simulink library "Model_GridElem_Arc_Fault"  (R2022b)
settings: Solver=VariableStepAuto  StartTime=0.0  StopTime=10.0  RelTol=1e-3
undefined symbols (not defined in the file): DiscIntNeverNeededParam
libraries: powerlib x220, spsVariableResistorLib x3, spsControlledVoltageSourceLib x3, spsGroundLib x1, spsThreePhaseVIMeasurementLib x1
(part 1 of 2)
settings Model: Creator=winkens  LastModifiedBy=winkens
settings SolverCC: AlgebraicLoopSolver=TrustRegion
settings DebuggingCC: UnconnectedInputMsg=warning  UnconnectedOutputMsg=warning  UnconnectedLineMsg=warning  SFMachineParentedDataDiag=warning
settings ModelReferenceCC: EnableRefExpFcnMdlSchedulingChecks=on
settings RTWCC: DLArmComputeVersion=19.05

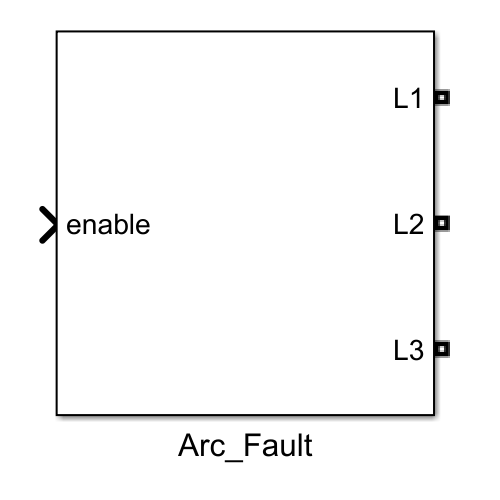
[thumbnail: Simulink's stored preview of the top-level diagram]
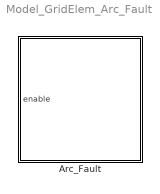
== system Model_GridElem_Arc_Fault ==
  Arc_Fault : Subsystem  mask{faultType=L1<>GRD | L2<>GRD | L3<>GRD, arcModel=Resistor, R_arc=0, ArcCurve_i=[-90 -100 -105 -110 -120 -150 -200 0 200 150 120 110 105 100 90], ArcCurve_v=[-2000 -1000 -500 -400 -300 -200 -100 0 100 200 300 400 500 1000 2000], Mayr_P_0=10e3, Mayr_T=100e-6, Mayr_G_max=100, Mayr_G_min=1, Cassie_V_0=150, Cassie_T=200e-6, Cassie_G_max=100, Cassie_G_min=1}
      mask prompts: faultType "Fault Type:"; arcModel "Arc Model:"; R_arc "Arc Resistance [Ohm]:"; ArcCurve_i "Current vector [A]:"; ArcCurve_v "Voltage vector [V]:"; Mayr_P_0 "Constant heat loss [W]:"; Mayr_T "Time Constant [s]:"; Mayr_G_max "Maximum Arc Conductance [S]:"; Mayr_G_min "Minimum Arc Conductance [S]:"; Cassie_V_0 "Cassie Voltage Level V_0 [V]:"; Cassie_T "Time Constant [s]:"; Cassie_G_max "Maximum Arc Conductance [S]:"; Cassie_G_min "Minimum Arc Conductance [S]:"
      mask TypeOptions faultType: L1<>GRD | L2<>GRD | L3<>GRD | L1<>L2 | L2<>L3 | L3<>L1 | L1<>L2 | L2<>L3 | L1<>GRD | L2<>GRD | L1<>L2 | L1<>GRD
      mask Callback faultType:
      | msk = Simulink.Mask.get(gcb);
      | p = msk.Parameters;
      | if strcmp(get_param(gcb, 'faultType'), 'L1<>GRD | L2<>GRD | L3<>GRD')
      |     %L1<>GRD | L2<>GRD | L3<>GRD
      |     set_param([gcb '/Fault_Model/Resistor/Electric_Model'],'LabelModeActivechoice','L1G_L2G_L3G');
      |     set_param([gcb '/Fault_Model/Arc_Characteristic_Curve/Electric_Model'],'LabelModeActivechoice','L1G_L2G_L3G');
      |     set_param([gcb '/Fault_Model/Mayr_Model/Electric_Model'],'LabelModeActivechoice','L1G_L2G_L3G');
      |     set_param([gcb '/Fault_Model/Cassie_Model/Electric_Model'],'LabelModeActivechoice','L1G_L2G_L3G');
      | 
      | elseif strcmp(get_param(gcb, 'faultType'), 'L1<>L2 | L2<>L3 | L3<>L1')
      |     %L1<>L2 | L2<>L3 | L3<>L1
      |     set_param([gcb '/Fault_Model/Resistor/Electric_Model'],'LabelModeActivechoice','L1L2_L2L3_L3L1');
      |     set_param([gcb '/Fault_Model/Arc_Characteristic_Curve/Electric_Model'],'LabelModeActivechoice','L1L2_L2L3_L3L1');
      |     set_param([gcb '/Fault_Model/Mayr_Model/Electric_Model'],'LabelModeActivechoice','L1L2_L2L3_L3L1');
      |     set_param([gcb '/Fault_Model/Cassie_Model/Electric_Model'],'LabelModeActivechoice','L1L2_L2L3_L3L1');
      | 
      | elseif strcmp(get_param(gcb, 'faultType'), 'L1<>GRD | L2<>GRD')
      |     %L1<>GRD | L2<>GRD
      |     set_param([gcb '/Fault_Model/Resistor/Electric_Model'],'LabelModeActivechoice','L1G_L2G');
      |     set_param([gcb '/Fault_Model/Arc_Characteristic_Curve/Electric_Model'],'LabelModeActivechoice','L1G_L2G');
      |     set_param([gcb '/Fault_Model/Mayr_Model/Electric_Model'],'LabelModeActivechoice','L1G_L2G');
      |     set_param([gcb '/Fault_Model/Cassie_Model/Electric_Model'],'LabelModeActivechoice','L1G_L2G');
      | 
      | elseif strcmp(get_param(gcb, 'faultType'), 'L1<>L2 | L2<>L3')
      |     %L1<>L2 | L2<>L3
      |     set_param([gcb '/Fault_Model/Resistor/Electric_Model'],'LabelModeActivechoice','L1L2_L2L3');
      |     set_param([gcb '/Fault_Model/Arc_Characteristic_Curve/Electric_Model'],'LabelModeActivechoice','L1L2_L2L3');
      |     set_param([gcb '/Fault_Model/Mayr_Model/Electric_Model'],'LabelModeActivechoice','L1L2_L2L3');
      |     set_param([gcb '/Fault_Model/Cassie_Model/Electric_Model'],'LabelModeActivechoice','L1L2_L2L3');
      | 
      | elseif strcmp(get_param(gcb, 'faultType'), 'L1<>GRD')
      |     %L1<>GRD
      |     set_param([gcb '/Fault_Model/Resistor/Electric_Model'],'LabelModeActivechoice','L1G');
      |     set_param([gcb '/Fault_Model/Arc_Characteristic_Curve/Electric_Model'],'LabelModeActivechoice','L1G');
      |     set_param([gcb '/Fault_Model/Mayr_Model/Electric_Model'],'LabelModeActivechoice','L1G');
      |     set_param([gcb '/Fault_Model/Cassie_Model/Electric_Model'],'LabelModeActivechoice','L1G');
      | 
      | elseif strcmp(get_param(gcb, 'faultType'), 'L1<>L2')
      |     %L1<>L2
      |     set_param([gcb '/Fault_Model/Resistor/Electric_Model'],'LabelModeActivechoice','L1L2');
      |     set_param([gcb '/Fault_Model/Arc_Characteristic_Curve/Electric_Model'],'LabelModeActivechoice','L1L2');
      |     set_param([gcb '/Fault_Model/Mayr_Model/Electric_Model'],'LabelModeActivechoice','L1L2');
      |     set_param([gcb '/Fault_Model/Cassie_Model/Electric_Model'],'LabelModeActivechoice','L1L2');
      | end
      mask TypeOptions arcModel: Resistor | Arc Characteristic Curve | Mayr Model | Cassie Model
      mask Callback arcModel:
      | msk = Simulink.Mask.get(gcb);
      | p = msk.Parameters;
      | if strcmp(get_param(gcb, 'arcModel'), 'Resistor')
      |     %Resistor
      |     msk.getDialogControl('boxResistor').Visible = 'on';
      |     msk.getDialogControl('boxArcCurve').Visible = 'off';
      |     msk.getDialogControl('boxMayr').Visible = 'off';
      |     msk.getDialogControl('boxCassie').Visible = 'off';
      |     set_param([gcb '/Fault_Model'],'LabelModeActivechoice','Resistor');
      | elseif strcmp(get_param(gcb, 'arcModel'), 'Arc Characteristic Curve')
      |     %Arc Curve
      |     msk.getDialogControl('boxResistor').Visible = 'off';
      |     msk.getDialogControl('boxArcCurve').Visible = 'on';
      |     msk.getDialogControl('boxMayr').Visible = 'off';
      |     msk.getDialogControl('boxCassie').Visible = 'off';
      |     set_param([gcb '/Fault_Model'],'LabelModeActivechoice','Arc_Characteristic_Curve');
      | elseif strcmp(get_param(gcb, 'arcModel'), 'Mayr Model')
      |     %Mayr
      |     msk.getDialogControl('boxResistor').Visible = 'off';
      |     msk.getDialogControl('boxArcCurve').Visible = 'off';
      |     msk.getDialogControl('boxMayr').Visible = 'on';
      |     msk.getDialogControl('boxCassie').Visible = 'off';
      |     set_param([gcb '/Fault_Model'],'LabelModeActivechoice','Mayr_Model');
      | elseif strcmp(get_param(gcb, 'arcModel'), 'Cassie Model')
      |     %Cassie
      |     msk.getDialogControl('boxResistor').Visible = 'off';
      |     msk.getDialogControl('boxArcCurve').Visible = 'off';
      |     msk.getDialogControl('boxMayr').Visible = 'off';
      |     msk.getDialogControl('boxCassie').Visible = 'on';
      |     set_param([gcb '/Fault_Model'],'LabelModeActivechoice','Cassie_Model');
      | end
      mask DialogControl DescGroupVar Prompt: Arc Fault
      mask DialogControl DescTextVar Prompt: Fault model for detailed representation of the arc behavior.
      mask DialogControl boxParam Prompt: Parameters
      mask DialogControl boxResistor Prompt: Resistor Parameters
      mask DialogControl boxArcCurve Prompt: Arc Characteristic Curve Parameters
      mask DialogControl textArcCurve Prompt: The arc characteristic curve is modeled as a lookup table. The voltage and current vectors define the characteristic points of the curve.
      mask DialogControl boxMayr Prompt: Mayr Parameters
      mask DialogControl boxCassie Prompt: Cassie Parameters

== system Model_GridElem_Arc_Fault/Arc_Fault ==
  enable : Inport
  Fault_Model : Subsystem  Variant=on  VariantControlMode=label  VariantControl=Choice  LabelModeActiveChoice=Resistor
  L1 : PMIOPort  Side=Right
  L2 : PMIOPort  Port=2  Side=Right
  L3 : PMIOPort  Port=3  Side=Right
  wires:
  enable/1 -> Fault_Model/1(enable)
  connections:
  Fault_Model/RConn1 -- L1/RConn1
  Fault_Model/RConn2 -- L2/RConn1
  Fault_Model/RConn3 -- L3/RConn1

== system Model_GridElem_Arc_Fault/Arc_Fault/Fault_Model ==
  enable : Inport
  Arc_Characteristic_Curve : Subsystem  VariantControl=Arc_Characteristic_Curve
  Cassie_Model : Subsystem  VariantControl=Cassie_Model
  Mayr_Model : Subsystem  VariantControl=Mayr_Model
  Resistor : Subsystem  VariantControl=Resistor
  L1 : PMIOPort  Side=Right
  L2 : PMIOPort  Port=2  Side=Right
  L3 : PMIOPort  Port=3  Side=Right

== system Model_GridElem_Arc_Fault/Arc_Fault/Fault_Model/Arc_Characteristic_Curve ==
  enable : Inport
  Arc_Voltage_Calculation : Subsystem
  Electric_Model : Subsystem  Variant=on  VariantControlMode=label  LabelModeActiveChoice=L1G_L2G_L3G
  Terminator : Terminator
  L1 : PMIOPort  Side=Right
  L2 : PMIOPort  Port=2  Side=Right
  L3 : PMIOPort  Port=3  Side=Right
  wires:
  enable/1 -> Arc_Voltage_Calculation/3(enable)
  Electric_Model/3(v_arc_meas) -> Terminator/1
  Arc_Voltage_Calculation/3(v_arc) -> Electric_Model/3(v_arc)
  Arc_Voltage_Calculation/2(R_arc) -> Electric_Model/2(R_arc)
  Arc_Voltage_Calculation/1(R_block) -> Electric_Model/1(R_block)
  Electric_Model/1(numberOfArcs) -> Arc_Voltage_Calculation/1(numberOfArcs)
  Electric_Model/2(i_arc_meas) -> Arc_Voltage_Calculation/2(i_arc)
  connections:
  L2/RConn1 -- Electric_Model/RConn2
  L3/RConn1 -- Electric_Model/RConn3
  L1/RConn1 -- Electric_Model/RConn1

== system Model_GridElem_Arc_Fault/Arc_Fault/Fault_Model/Cassie_Model ==
  enable : Inport
  Cassie_Arc_Model : Subsystem
  Electric_Model : Subsystem  Variant=on  VariantControlMode=label  LabelModeActiveChoice=L1G_L2G_L3G
  Terminator : Terminator
  L1 : PMIOPort  Side=Right
  L2 : PMIOPort  Port=2  Side=Right
  L3 : PMIOPort  Port=3  Side=Right
  wires:
  enable/1 -> Cassie_Arc_Model/3(enable)
  Electric_Model/2(i_arc_meas) -> Terminator/1
  Cassie_Arc_Model/2(R_arc) -> Electric_Model/2(R_arc)
  Cassie_Arc_Model/1(R_block) -> Electric_Model/1(R_block)
  Cassie_Arc_Model/3(v_arc) -> Electric_Model/3(v_arc)
  Electric_Model/1(numberOfArcs) -> Cassie_Arc_Model/1(numberOfArcs)
  Electric_Model/3(v_arc_meas) -> Cassie_Arc_Model/2(v_arc_meas)
  connections:
  L1/RConn1 -- Electric_Model/RConn1
  L2/RConn1 -- Electric_Model/RConn2
  L3/RConn1 -- Electric_Model/RConn3

== system Model_GridElem_Arc_Fault/Arc_Fault/Fault_Model/Mayr_Model ==
  enable : Inport
  Electric_Model : Subsystem  Variant=on  VariantControlMode=label  LabelModeActiveChoice=L1G_L2G_L3G
  Mayr_Arc_Model : Subsystem
  Terminator : Terminator
  L1 : PMIOPort  Side=Right
  L2 : PMIOPort  Port=2  Side=Right
  L3 : PMIOPort  Port=3  Side=Right
  wires:
  enable/1 -> Mayr_Arc_Model/3(enable)
  Electric_Model/3(v_arc_meas) -> Terminator/1
  Mayr_Arc_Model/2(R_arc) -> Electric_Model/2(R_arc)
  Mayr_Arc_Model/1(R_block) -> Electric_Model/1(R_block)
  Mayr_Arc_Model/3(v_arc) -> Electric_Model/3(v_arc)
  Electric_Model/1(numberOfArcs) -> Mayr_Arc_Model/1(numberOfArcs)
  Electric_Model/2(i_arc_meas) -> Mayr_Arc_Model/2(i_arc)
  connections:
  L2/RConn1 -- Electric_Model/RConn2
  L3/RConn1 -- Electric_Model/RConn3
  L1/RConn1 -- Electric_Model/RConn1

== system Model_GridElem_Arc_Fault/Arc_Fault/Fault_Model/Resistor ==
  enable : Inport
  Constant : Constant  Value=0
  Constant1 : Constant  Value=1e7
  Constant2 : Constant  Value=0
  Constant3 : Constant  Value=R_arc
  Divide1 : Product  Inputs=**
  Divide2 : Product  Inputs=**
  Divide3 : Product  Inputs=**
  Electric_Model : Subsystem  Variant=on  VariantControlMode=label  LabelModeActiveChoice=L1G_L2G_L3G
  Switch : Switch  Criteria=u2 > Threshold  SaturateOnIntegerOverflow=off  InputSameDT=off
  Terminator : Terminator
  Terminator1 : Terminator
  L1 : PMIOPort  Side=Right
  L2 : PMIOPort  Port=2  Side=Right
  L3 : PMIOPort  Port=3  Side=Right
  wires:
  enable/1 -> Switch/2
  Constant/1 -> Switch/1
  Constant1/1 -> Switch/3
  Electric_Model/3(v_arc_meas) -> Terminator/1
  Divide3/1 -> Electric_Model/3(v_arc)
  Divide2/1 -> Electric_Model/2(R_arc)
  Divide1/1 -> Electric_Model/1(R_block)
  Constant2/1 -> Divide3/1
  Constant3/1 -> Divide2/1
  Switch/1 -> Divide1/1
  Electric_Model/1(numberOfArcs) -> Divide3/2, Divide2/2, Divide1/2
  Electric_Model/2(i_arc_meas) -> Terminator1/1
  connections:
  Electric_Model/RConn2 -- L2/RConn1
  Electric_Model/RConn1 -- L1/RConn1
  Electric_Model/RConn3 -- L3/RConn1

== system Model_GridElem_Arc_Fault/Arc_Fault/Fault_Model/Arc_Characteristic_Curve/Arc_Voltage_Calculation ==
  numberOfArcs : Inport
  i_arc : Inport  Port=2
  enable : Inport  Port=3
  Constant : Constant  Value=1e7
  Constant1 : Constant  Value=0
  Constant2 : Constant  Value=0
  Constant3 : Constant  Value=0
  Divide{,1..3} (4 alike) : Product  Inputs=**
  Nonlinear_Resistor_Curve : Subsystem
  Switch : Switch  Criteria=u2 > Threshold  SaturateOnIntegerOverflow=off  InputSameDT=off
  Switch1 : Switch  Criteria=u2 > Threshold  SaturateOnIntegerOverflow=off  InputSameDT=off
  Unit Delay1 : UnitDelay  SampleTime=-1  HasFrameUpgradeWarning=on
  R_block : Outport
  R_arc : Outport  Port=2
  v_arc : Outport  Port=3
  wires:
  i_arc/1 -> Unit Delay1/1
  Nonlinear_Resistor_Curve/1(v_arc) -> Switch1/1
  Switch/1 -> R_block/1
  enable/1 -> Nonlinear_Resistor_Curve/Enable, Switch1/2, Switch/2
  Unit Delay1/1 -> Nonlinear_Resistor_Curve/1(i_arc)
  Switch1/1 -> v_arc/1
  Divide2/1 -> R_arc/1
  Divide/1 -> Switch/1
  Constant/1 -> Divide1/1
  Divide1/1 -> Switch/3
  Constant1/1 -> Divide/1
  Constant3/1 -> Divide2/1
  Constant2/1 -> Divide3/1
  Divide3/1 -> Switch1/3
  numberOfArcs/1 -> Divide3/2, Divide2/2, Divide1/2, Divide/2

== system Model_GridElem_Arc_Fault/Arc_Fault/Fault_Model/Arc_Characteristic_Curve/Electric_Model ==
  R_block : Inport
  R_arc : Inport  Port=2
  v_arc : Inport  Port=3
  L1G : Subsystem  VariantControl=L1G
  L1G_L2G : Subsystem  VariantControl=L1G_L2G
  L1G_L2G_L3G : Subsystem  VariantControl=L1G_L2G_L3G
  L1L2 : Subsystem  VariantControl=L1L2
  L1L2_L2L3 : Subsystem  VariantControl=L1L2_L2L3
  L1L2_L2L3_L3L1 : Subsystem  VariantControl=L1L2_L2L3_L3L1
  L1 : PMIOPort  Side=Right
  L2 : PMIOPort  Port=2  Side=Right
  L3 : PMIOPort  Port=3  Side=Right
  numberOfArcs : Outport
  i_arc_meas : Outport  Port=2
  v_arc_meas : Outport  Port=3

== system Model_GridElem_Arc_Fault/Arc_Fault/Fault_Model/Cassie_Model/Cassie_Arc_Model ==
  numberOfArcs : Inport
  v_arc_meas : Inport  Port=2
  enable : Inport  Port=3
  Arc_Equations : Subsystem
  Constant : Constant  Value=0
  Constant1 : Constant  Value=0
  Constant2 : Constant  Value=1e7
  Constant3 : Constant  Value=0
  Divide{,1..3} (4 alike) : Product  Inputs=**
  Switch : Switch  Criteria=u2 > Threshold  SaturateOnIntegerOverflow=off  InputSameDT=off
  Switch1 : Switch  Criteria=u2 > Threshold  SaturateOnIntegerOverflow=off  InputSameDT=off
  Unit Delay : UnitDelay  SampleTime=-1  HasFrameUpgradeWarning=on
  Unit Delay1 : UnitDelay  SampleTime=-1  HasFrameUpgradeWarning=on
  R_block : Outport
  R_arc : Outport  Port=2
  v_arc : Outport  Port=3
  wires:
  enable/1 -> Arc_Equations/1(enable), Unit Delay/1, Arc_Equations/Enable
  v_arc_meas/1 -> Unit Delay1/1
  Arc_Equations/1(R_arc) -> Switch/1
  Switch/1 -> R_arc/1
  Unit Delay/1 -> Switch1/2, Switch/2
  Unit Delay1/1 -> Arc_Equations/3(v_abc)
  Switch1/1 -> R_block/1
  Divide/1 -> Switch1/1
  Divide1/1 -> Switch1/3
  Divide2/1 -> Switch/3
  Divide3/1 -> v_arc/1
  Constant/1 -> Divide2/1
  Constant1/1 -> Divide/1
  Constant2/1 -> Divide1/1
  Constant3/1 -> Divide3/1
  numberOfArcs/1 -> Arc_Equations/2(numberOfArcs), Divide3/2, Divide2/2, Divide1/2, Divide/2

== system Model_GridElem_Arc_Fault/Arc_Fault/Fault_Model/Cassie_Model/Electric_Model ==
  R_block : Inport
  R_arc : Inport  Port=2
  v_arc : Inport  Port=3
  L1G : Subsystem  VariantControl=L1G
  L1G_L2G : Subsystem  VariantControl=L1G_L2G
  L1G_L2G_L3G : Subsystem  VariantControl=L1G_L2G_L3G
  L1L2 : Subsystem  VariantControl=L1L2
  L1L2_L2L3 : Subsystem  VariantControl=L1L2_L2L3
  L1L2_L2L3_L3L1 : Subsystem  VariantControl=L1L2_L2L3_L3L1
  L1 : PMIOPort  Side=Right
  L2 : PMIOPort  Port=2  Side=Right
  L3 : PMIOPort  Port=3  Side=Right
  numberOfArcs : Outport
  i_arc_meas : Outport  Port=2
  v_arc_meas : Outport  Port=3

== system Model_GridElem_Arc_Fault/Arc_Fault/Fault_Model/Mayr_Model/Electric_Model ==
  R_block : Inport
  R_arc : Inport  Port=2
  v_arc : Inport  Port=3
  L1G : Subsystem  VariantControl=L1G
  L1G_L2G : Subsystem  VariantControl=L1G_L2G
  L1G_L2G_L3G : Subsystem  VariantControl=L1G_L2G_L3G
  L1L2 : Subsystem  VariantControl=L1L2
  L1L2_L2L3 : Subsystem  VariantControl=L1L2_L2L3
  L1L2_L2L3_L3L1 : Subsystem  VariantControl=L1L2_L2L3_L3L1
  L1 : PMIOPort  Side=Right
  L2 : PMIOPort  Port=2  Side=Right
  L3 : PMIOPort  Port=3  Side=Right
  numberOfArcs : Outport
  i_arc_meas : Outport  Port=2
  v_arc_meas : Outport  Port=3

== system Model_GridElem_Arc_Fault/Arc_Fault/Fault_Model/Mayr_Model/Mayr_Arc_Model ==
  numberOfArcs : Inport
  i_arc : Inport  Port=2
  enable : Inport  Port=3
  Arc_Equations : Subsystem
  Constant : Constant  Value=1e7
  Constant1 : Constant  Value=0
  Constant2 : Constant  Value=0
  Constant3 : Constant  Value=0
  Divide{,1..3} (4 alike) : Product  Inputs=**
  Switch : Switch  Criteria=u2 > Threshold  SaturateOnIntegerOverflow=off  InputSameDT=off
  Switch1 : Switch  Criteria=u2 > Threshold  SaturateOnIntegerOverflow=off  InputSameDT=off
  Unit Delay : UnitDelay  SampleTime=-1  HasFrameUpgradeWarning=on
  Unit Delay1 : UnitDelay  SampleTime=-1  HasFrameUpgradeWarning=on
  R_block : Outport
  R_arc : Outport  Port=2
  v_arc : Outport  Port=3
  wires:
  enable/1 -> Arc_Equations/1(enable), Unit Delay/1, Arc_Equations/Enable
  i_arc/1 -> Unit Delay1/1
  Arc_Equations/1(R_arc) -> Switch/1
  Constant/1 -> Divide1/1
  Switch/1 -> R_arc/1
  Unit Delay/1 -> Switch1/2, Switch/2
  Unit Delay1/1 -> Arc_Equations/3(i_abc)
  Switch1/1 -> R_block/1
  Divide3/1 -> v_arc/1
  Divide2/1 -> Switch/3
  Divide1/1 -> Switch1/3
  Divide/1 -> Switch1/1
  Constant1/1 -> Divide/1
  Constant2/1 -> Divide2/1
  Constant3/1 -> Divide3/1
  numberOfArcs/1 -> Arc_Equations/2(numberOfArcs), Divide3/2, Divide2/2, Divide1/2, Divide/2

== system Model_GridElem_Arc_Fault/Arc_Fault/Fault_Model/Resistor/Electric_Model ==
  R_block : Inport
  R_arc : Inport  Port=2
  v_arc : Inport  Port=3
  L1G : Subsystem  VariantControl=L1G
  L1G_L2G : Subsystem  VariantControl=L1G_L2G
  L1G_L2G_L3G : Subsystem  VariantControl=L1G_L2G_L3G
  L1L2 : Subsystem  VariantControl=L1L2
  L1L2_L2L3 : Subsystem  VariantControl=L1L2_L2L3
  L1L2_L2L3_L3L1 : Subsystem  VariantControl=L1L2_L2L3_L3L1
  L1 : PMIOPort  Side=Right
  L2 : PMIOPort  Port=2  Side=Right
  L3 : PMIOPort  Port=3  Side=Right
  numberOfArcs : Outport
  i_arc_meas : Outport  Port=2
  v_arc_meas : Outport  Port=3

== system Model_GridElem_Arc_Fault/Arc_Fault/Fault_Model/Arc_Characteristic_Curve/Arc_Voltage_Calculation/Nonlinear_Resistor_Curve ==
  i_arc : Inport
  Enable : EnablePort
  1-D Lookup Table : Lookup_n-D  NumberOfTableDimensions=1  BreakpointsForDimension1=ArcCurve_v  BreakpointsForDimension2=[-2000 - 1000 -500 -400 -300 -200 -100 0 100 200 300 400 500 1000 2000]  BreakpointsForDimension3=[-2000 - 1000 -500 -400 -300 -200 -100 0 100 200 300 400 500 1000 2000]  Table=ArcCurve_i  ExtrapMethod=Clip  UseLastTableValue=on  InternalRulePriority=Speed  RndMeth=Simplest
  v_arc : Outport
  wires:
  1-D Lookup Table/1 -> v_arc/1
  i_arc/1 -> 1-D Lookup Table/1

== system Model_GridElem_Arc_Fault/Arc_Fault/Fault_Model/Arc_Characteristic_Curve/Electric_Model/L1G ==
  R_block : Inport
  R_arc : Inport  Port=2
  v_arc : Inport  Port=3
  Add : Sum  Inputs=++|
  Arc_Resistance_L1G : powerlib/Elements/Variable Resistor  Rabsmin=1e-6
  Arc_Voltage_L1G : powerlib/Electrical Sources/Controlled Voltage Source  Initialize=on  Source_Type=AC  Amplitude=0  Phase=0  Frequency=0  Measurements=None
  Constant : Constant
  Current Measurement : powerlib/Measurements/Current Measurement  PhasorSimulation=off  OutputType=Complex  PSBequivalent=0
  Ground{,1..3} (4 alike) : powerlib/Elements/Ground  LConnTagsString=a
  Terminator : Terminator
  Terminator1 : Terminator
  Voltage Measurement : powerlib/Measurements/Voltage Measurement  PhasorSimulation=off  OutputType=Complex  PSBequivalent=0
  Voltage Measurement1 : powerlib/Measurements/Voltage Measurement  PhasorSimulation=off  OutputType=Complex  PSBequivalent=0
  Voltage Measurement2 : powerlib/Measurements/Voltage Measurement  PhasorSimulation=off  OutputType=Complex  PSBequivalent=0
  L1 : PMIOPort  Side=Right
  L2 : PMIOPort  Port=2  Side=Right
  L3 : PMIOPort  Port=3  Side=Right
  numberOfArcs : Outport
  i_arc_meas : Outport  Port=2
  v_arc_meas : Outport  Port=3
  wires:
  Voltage Measurement/1 -> v_arc_meas/1
  Voltage Measurement2/1 -> Terminator/1
  v_arc/1 -> Arc_Voltage_L1G/1
  Current Measurement/1 -> i_arc_meas/1
  Voltage Measurement1/1 -> Terminator1/1
  R_arc/1 -> Add/2
  R_block/1 -> Add/1
  Add/1 -> Arc_Resistance_L1G/1
  Constant/1 -> numberOfArcs/1
  connections:
  Current Measurement/RConn1 -- Arc_Resistance_L1G/RConn1 -- Voltage Measurement/LConn1
  Ground/LConn1 -- Arc_Voltage_L1G/LConn1
  Current Measurement/LConn1 -- L1/RConn1
  Voltage Measurement2/LConn1 -- L3/RConn1
  Ground1/LConn1 -- Voltage Measurement/LConn2
  Voltage Measurement2/LConn2 -- Ground3/LConn1
  Arc_Voltage_L1G/RConn1 -- Arc_Resistance_L1G/LConn1
  Voltage Measurement1/LConn1 -- L2/RConn1
  Voltage Measurement1/LConn2 -- Ground2/LConn1

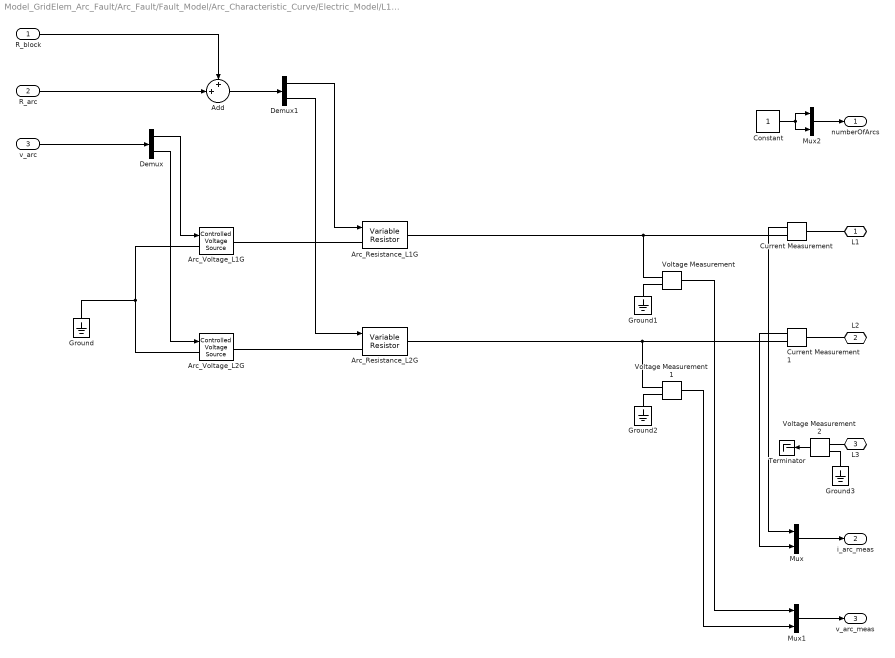
== system Model_GridElem_Arc_Fault/Arc_Fault/Fault_Model/Arc_Characteristic_Curve/Electric_Model/L1G_L2G ==
  R_block : Inport
  R_arc : Inport  Port=2
  v_arc : Inport  Port=3
  Add : Sum  Inputs=++|
  Arc_Resistance_L1G : powerlib/Elements/Variable Resistor  Rabsmin=1e-6
  Arc_Resistance_L2G : powerlib/Elements/Variable Resistor  Rabsmin=1e-6
  Arc_Voltage_L1G : powerlib/Electrical Sources/Controlled Voltage Source  Initialize=on  Source_Type=AC  Amplitude=0  Phase=0  Frequency=0  Measurements=None
  Arc_Voltage_L2G : powerlib/Electrical Sources/Controlled Voltage Source  Initialize=on  Source_Type=AC  Amplitude=0  Phase=0  Frequency=0  Measurements=None
  Constant : Constant
  Current Measurement : powerlib/Measurements/Current Measurement  PhasorSimulation=off  OutputType=Complex  PSBequivalent=0
  Current Measurement1 : powerlib/Measurements/Current Measurement  PhasorSimulation=off  OutputType=Complex  PSBequivalent=0
  Demux : Demux  Outputs=2
  Demux1 : Demux  Outputs=2
  Ground{,1..3} (4 alike) : powerlib/Elements/Ground  LConnTagsString=a
  Mux : Mux  Inputs=2
  Mux1 : Mux  Inputs=2
  Mux2 : Mux  Inputs=2
  Terminator : Terminator
  Voltage Measurement : powerlib/Measurements/Voltage Measurement  PhasorSimulation=off  OutputType=Complex  PSBequivalent=0
  Voltage Measurement1 : powerlib/Measurements/Voltage Measurement  PhasorSimulation=off  OutputType=Complex  PSBequivalent=0
  Voltage Measurement2 : powerlib/Measurements/Voltage Measurement  PhasorSimulation=off  OutputType=Complex  PSBequivalent=0
  L1 : PMIOPort  Side=Right
  L2 : PMIOPort  Port=2  Side=Right
  L3 : PMIOPort  Port=3  Side=Right
  numberOfArcs : Outport
  i_arc_meas : Outport  Port=2
  v_arc_meas : Outport  Port=3
  wires:
  Demux/1 -> Arc_Voltage_L1G/1
  v_arc/1 -> Demux/1
  Demux1/1 -> Arc_Resistance_L1G/1
  Demux1/2 -> Arc_Resistance_L2G/1
  Demux/2 -> Arc_Voltage_L2G/1
  Mux/1 -> i_arc_meas/1
  Mux1/1 -> v_arc_meas/1
  Current Measurement/1 -> Mux/1
  Current Measurement1/1 -> Mux/2
  Voltage Measurement/1 -> Mux1/1
  Voltage Measurement1/1 -> Mux1/2
  Voltage Measurement2/1 -> Terminator/1
  R_arc/1 -> Add/2
  Add/1 -> Demux1/1
  R_block/1 -> Add/1
  Mux2/1 -> numberOfArcs/1
  Constant/1 -> Mux2/2, Mux2/1
  connections:
  Ground/LConn1 -- Arc_Voltage_L2G/LConn1 -- Arc_Voltage_L1G/LConn1
  Voltage Measurement2/LConn1 -- L3/RConn1
  Arc_Voltage_L2G/RConn1 -- Arc_Resistance_L2G/LConn1
  Arc_Voltage_L1G/RConn1 -- Arc_Resistance_L1G/LConn1
  Current Measurement/RConn1 -- Arc_Resistance_L1G/RConn1 -- Voltage Measurement/LConn1
  Current Measurement/LConn1 -- L1/RConn1
  Current Measurement1/RConn1 -- Arc_Resistance_L2G/RConn1 -- Voltage Measurement1/LConn1
  Current Measurement1/LConn1 -- L2/RConn1
  Ground1/LConn1 -- Voltage Measurement/LConn2
  Ground2/LConn1 -- Voltage Measurement1/LConn2
  Voltage Measurement2/LConn2 -- Ground3/LConn1

== system Model_GridElem_Arc_Fault/Arc_Fault/Fault_Model/Arc_Characteristic_Curve/Electric_Model/L1G_L2G_L3G ==
  R_block : Inport
  R_arc : Inport  Port=2
  v_arc : Inport  Port=3
  Add : Sum  Inputs=++|
  Arc_Resistance_L1G : powerlib/Elements/Variable Resistor  Rabsmin=1e-6
  Arc_Resistance_L2G : powerlib/Elements/Variable Resistor  Rabsmin=1e-6
  Arc_Resistance_L3G : powerlib/Elements/Variable Resistor  Rabsmin=1e-6
  Arc_Voltage_L1G : powerlib/Electrical Sources/Controlled Voltage Source  Initialize=on  Source_Type=AC  Amplitude=0  Phase=0  Frequency=0  Measurements=None
  Arc_Voltage_L2G : powerlib/Electrical Sources/Controlled Voltage Source  Initialize=on  Source_Type=AC  Amplitude=0  Phase=0  Frequency=0  Measurements=None
  Arc_Voltage_L3G : powerlib/Electrical Sources/Controlled Voltage Source  Initialize=on  Source_Type=AC  Amplitude=0  Phase=0  Frequency=0  Measurements=None
  Constant : Constant
  Demux : Demux  Outputs=3
  Demux1 : Demux  Outputs=3
  Ground : powerlib/Elements/Ground  LConnTagsString=a
  Mux : Mux  Inputs=3
  Three-Phase V-I Measurement : powerlib/Measurements/Three-Phase V-I Measurement  VoltageMeasurement=phase-to-ground  SetLabelV=off  LabelV=Vabc  Vpu=off  VpuLL=off  CurrentMeasurement=yes  SetLabelI=off  LabelI=Iabc  Ipu=off  Pbase=100e6  Vbase=500e3  OutputType=Complex  PhasorSimulation=off  PSBequivalent=0
  L1 : PMIOPort  Side=Right
  L2 : PMIOPort  Port=2  Side=Right
  L3 : PMIOPort  Port=3  Side=Right
  numberOfArcs : Outport
  i_arc_meas : Outport  Port=2
  v_arc_meas : Outport  Port=3
  wires:
  v_arc/1 -> Demux/1
  Three-Phase V-I Measurement/2 -> i_arc_meas/1
  Three-Phase V-I Measurement/1 -> v_arc_meas/1
  Demux/3 -> Arc_Voltage_L3G/1
  Demux/2 -> Arc_Voltage_L2G/1
  Demux/1 -> Arc_Voltage_L1G/1
  Demux1/3 -> Arc_Resistance_L3G/1
  Demux1/2 -> Arc_Resistance_L2G/1
  Demux1/1 -> Arc_Resistance_L1G/1
  R_arc/1 -> Add/2
  Add/1 -> Demux1/1
  R_block/1 -> Add/1
  Mux/1 -> numberOfArcs/1
  Constant/1 -> Mux/3, Mux/1, Mux/2
  connections:
  Three-Phase V-I Measurement/RConn2 -- Arc_Resistance_L2G/RConn1
  Arc_Voltage_L1G/RConn1 -- Arc_Resistance_L1G/LConn1
  Arc_Voltage_L2G/RConn1 -- Arc_Resistance_L2G/LConn1
  Arc_Voltage_L3G/RConn1 -- Arc_Resistance_L3G/LConn1
  Arc_Voltage_L1G/LConn1 -- Arc_Voltage_L2G/LConn1 -- Arc_Voltage_L3G/LConn1 -- Ground/LConn1
  Arc_Resistance_L1G/RConn1 -- Three-Phase V-I Measurement/RConn1
  Arc_Resistance_L3G/RConn1 -- Three-Phase V-I Measurement/RConn3
  Three-Phase V-I Measurement/LConn1 -- L1/RConn1
  Three-Phase V-I Measurement/LConn2 -- L2/RConn1
  Three-Phase V-I Measurement/LConn3 -- L3/RConn1

== system Model_GridElem_Arc_Fault/Arc_Fault/Fault_Model/Arc_Characteristic_Curve/Electric_Model/L1L2 ==
  R_block : Inport
  R_arc : Inport  Port=2
  v_arc : Inport  Port=3
  Add : Sum  Inputs=++|
  Arc_Resistance_L1L2 : powerlib/Elements/Variable Resistor  Rabsmin=1e-6
  Arc_Voltage_L1L2 : powerlib/Electrical Sources/Controlled Voltage Source  Initialize=on  Source_Type=AC  Amplitude=0  Phase=0  Frequency=0  Measurements=None
  Constant : Constant
  Current Measurement : powerlib/Measurements/Current Measurement  PhasorSimulation=off  OutputType=Complex  PSBequivalent=0
  Ground : powerlib/Elements/Ground  LConnTagsString=a
  Terminator : Terminator
  Voltage Measurement : powerlib/Measurements/Voltage Measurement  PhasorSimulation=off  OutputType=Complex  PSBequivalent=0
  Voltage Measurement1 : powerlib/Measurements/Voltage Measurement  PhasorSimulation=off  OutputType=Complex  PSBequivalent=0
  L1 : PMIOPort  Side=Right
  L2 : PMIOPort  Port=2  Side=Right
  L3 : PMIOPort  Port=3  Side=Right
  numberOfArcs : Outport
  i_arc_meas : Outport  Port=2
  v_arc_meas : Outport  Port=3
  wires:
  Current Measurement/1 -> i_arc_meas/1
  Voltage Measurement/1 -> v_arc_meas/1
  v_arc/1 -> Arc_Voltage_L1L2/1
  Voltage Measurement1/1 -> Terminator/1
  R_arc/1 -> Add/2
  Add/1 -> Arc_Resistance_L1L2/1
  R_block/1 -> Add/1
  Constant/1 -> numberOfArcs/1
  connections:
  Current Measurement/RConn1 -- Arc_Resistance_L1L2/RConn1 -- Voltage Measurement/LConn1
  Voltage Measurement/LConn2 -- Arc_Voltage_L1L2/LConn1 -- L2/RConn1
  Current Measurement/LConn1 -- L1/RConn1
  Arc_Voltage_L1L2/RConn1 -- Arc_Resistance_L1L2/LConn1
  Voltage Measurement1/LConn1 -- L3/RConn1
  Voltage Measurement1/LConn2 -- Ground/LConn1

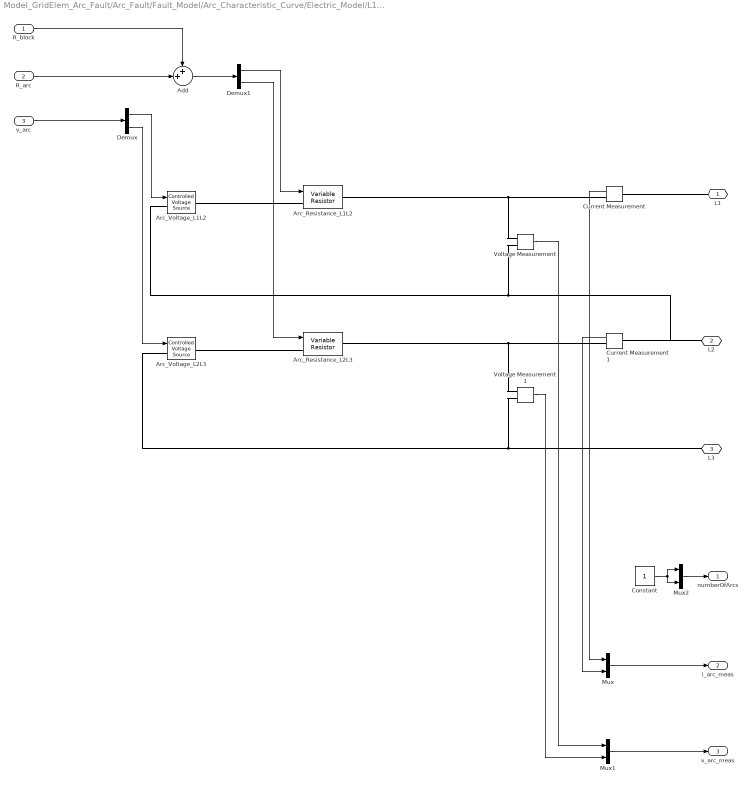
== system Model_GridElem_Arc_Fault/Arc_Fault/Fault_Model/Arc_Characteristic_Curve/Electric_Model/L1L2_L2L3 ==
  R_block : Inport
  R_arc : Inport  Port=2
  v_arc : Inport  Port=3
  Add : Sum  Inputs=++|
  Arc_Resistance_L1L2 : powerlib/Elements/Variable Resistor  Rabsmin=1e-6
  Arc_Resistance_L2L3 : powerlib/Elements/Variable Resistor  Rabsmin=1e-6
  Arc_Voltage_L1L2 : powerlib/Electrical Sources/Controlled Voltage Source  Initialize=on  Source_Type=AC  Amplitude=0  Phase=0  Frequency=0  Measurements=None
  Arc_Voltage_L2L3 : powerlib/Electrical Sources/Controlled Voltage Source  Initialize=on  Source_Type=AC  Amplitude=0  Phase=0  Frequency=0  Measurements=None
  Constant : Constant
  Current Measurement : powerlib/Measurements/Current Measurement  PhasorSimulation=off  OutputType=Complex  PSBequivalent=0
  Current Measurement1 : powerlib/Measurements/Current Measurement  PhasorSimulation=off  OutputType=Complex  PSBequivalent=0
  Demux : Demux  Outputs=2
  Demux1 : Demux  Outputs=2
  Mux : Mux  Inputs=2
  Mux1 : Mux  Inputs=2
  Mux2 : Mux  Inputs=2
  Voltage Measurement : powerlib/Measurements/Voltage Measurement  PhasorSimulation=off  OutputType=Complex  PSBequivalent=0
  Voltage Measurement1 : powerlib/Measurements/Voltage Measurement  PhasorSimulation=off  OutputType=Complex  PSBequivalent=0
  L1 : PMIOPort  Side=Right
  L2 : PMIOPort  Port=2  Side=Right
  L3 : PMIOPort  Port=3  Side=Right
  numberOfArcs : Outport
  i_arc_meas : Outport  Port=2
  v_arc_meas : Outport  Port=3
  wires:
  Current Measurement/1 -> Mux/1
  Mux/1 -> i_arc_meas/1
  Current Measurement1/1 -> Mux/2
  v_arc/1 -> Demux/1
  Demux/1 -> Arc_Voltage_L1L2/1
  Mux1/1 -> v_arc_meas/1
  Demux1/1 -> Arc_Resistance_L1L2/1
  Demux/2 -> Arc_Voltage_L2L3/1
  Voltage Measurement/1 -> Mux1/1
  Voltage Measurement1/1 -> Mux1/2
  Demux1/2 -> Arc_Resistance_L2L3/1
  Add/1 -> Demux1/1
  R_arc/1 -> Add/2
  R_block/1 -> Add/1
  Mux2/1 -> numberOfArcs/1
  Constant/1 -> Mux2/2, Mux2/1
  connections:
  Current Measurement/LConn1 -- L1/RConn1
  Current Measurement/RConn1 -- Arc_Resistance_L1L2/RConn1 -- Voltage Measurement/LConn1
  Voltage Measurement1/LConn2 -- Arc_Voltage_L2L3/LConn1 -- L3/RConn1
  Voltage Measurement/LConn2 -- Current Measurement1/LConn1 -- L2/RConn1 -- Arc_Voltage_L1L2/LConn1
  Current Measurement1/RConn1 -- Arc_Resistance_L2L3/RConn1 -- Voltage Measurement1/LConn1
  Arc_Voltage_L2L3/RConn1 -- Arc_Resistance_L2L3/LConn1
  Arc_Voltage_L1L2/RConn1 -- Arc_Resistance_L1L2/LConn1

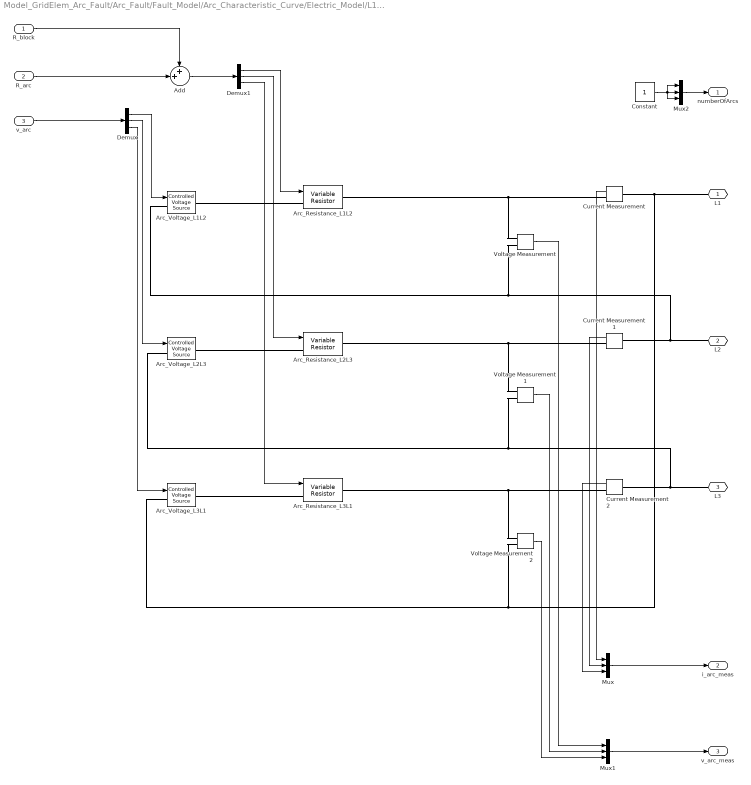
== system Model_GridElem_Arc_Fault/Arc_Fault/Fault_Model/Arc_Characteristic_Curve/Electric_Model/L1L2_L2L3_L3L1 ==
  R_block : Inport
  R_arc : Inport  Port=2
  v_arc : Inport  Port=3
  Add : Sum  Inputs=++|
  Arc_Resistance_L1L2 : powerlib/Elements/Variable Resistor  Rabsmin=1e-6
  Arc_Resistance_L2L3 : powerlib/Elements/Variable Resistor  Rabsmin=1e-6
  Arc_Resistance_L3L1 : powerlib/Elements/Variable Resistor  Rabsmin=1e-6
  Arc_Voltage_L1L2 : powerlib/Electrical Sources/Controlled Voltage Source  Initialize=on  Source_Type=AC  Amplitude=0  Phase=0  Frequency=0  Measurements=None
  Arc_Voltage_L2L3 : powerlib/Electrical Sources/Controlled Voltage Source  Initialize=on  Source_Type=AC  Amplitude=0  Phase=0  Frequency=0  Measurements=None
  Arc_Voltage_L3L1 : powerlib/Electrical Sources/Controlled Voltage Source  Initialize=on  Source_Type=AC  Amplitude=0  Phase=0  Frequency=0  Measurements=None
  Constant : Constant
  Current Measurement : powerlib/Measurements/Current Measurement  PhasorSimulation=off  OutputType=Complex  PSBequivalent=0
  Current Measurement1 : powerlib/Measurements/Current Measurement  PhasorSimulation=off  OutputType=Complex  PSBequivalent=0
  Current Measurement2 : powerlib/Measurements/Current Measurement  PhasorSimulation=off  OutputType=Complex  PSBequivalent=0
  Demux : Demux  Outputs=3
  Demux1 : Demux  Outputs=3
  Mux : Mux  Inputs=3
  Mux1 : Mux  Inputs=3
  Mux2 : Mux  Inputs=3
  Voltage Measurement : powerlib/Measurements/Voltage Measurement  PhasorSimulation=off  OutputType=Complex  PSBequivalent=0
  Voltage Measurement1 : powerlib/Measurements/Voltage Measurement  PhasorSimulation=off  OutputType=Complex  PSBequivalent=0
  Voltage Measurement2 : powerlib/Measurements/Voltage Measurement  PhasorSimulation=off  OutputType=Complex  PSBequivalent=0
  L1 : PMIOPort  Side=Right
  L2 : PMIOPort  Port=2  Side=Right
  L3 : PMIOPort  Port=3  Side=Right
  numberOfArcs : Outport
  i_arc_meas : Outport  Port=2
  v_arc_meas : Outport  Port=3
  wires:
  R_block/1 -> Add/1
  Demux1/3 -> Arc_Resistance_L3L1/1
  Demux/1 -> Arc_Voltage_L1L2/1
  v_arc/1 -> Demux/1
  Demux1/1 -> Arc_Resistance_L1L2/1
  Demux/3 -> Arc_Voltage_L3L1/1
  Demux1/2 -> Arc_Resistance_L2L3/1
  Demux/2 -> Arc_Voltage_L2L3/1
  Mux/1 -> i_arc_meas/1
  Mux1/1 -> v_arc_meas/1
  Current Measurement/1 -> Mux/1
  Current Measurement1/1 -> Mux/2
  Current Measurement2/1 -> Mux/3
  Voltage Measurement/1 -> Mux1/1
  Voltage Measurement1/1 -> Mux1/2
  Voltage Measurement2/1 -> Mux1/3
  Add/1 -> Demux1/1
  R_arc/1 -> Add/2
  Mux2/1 -> numberOfArcs/1
  Constant/1 -> Mux2/3, Mux2/1, Mux2/2
  connections:
  Arc_Voltage_L1L2/RConn1 -- Arc_Resistance_L1L2/LConn1
  Arc_Voltage_L3L1/RConn1 -- Arc_Resistance_L3L1/LConn1
  Arc_Voltage_L2L3/RConn1 -- Arc_Resistance_L2L3/LConn1
  Arc_Voltage_L3L1/LConn1 -- Voltage Measurement2/LConn2 -- L1/RConn1 -- Current Measurement/LConn1
  Arc_Voltage_L2L3/LConn1 -- Voltage Measurement1/LConn2 -- Current Measurement2/LConn1 -- L3/RConn1
  L2/RConn1 -- Arc_Voltage_L1L2/LConn1 -- Voltage Measurement/LConn2 -- Current Measurement1/LConn1
  Current Measurement/RConn1 -- Arc_Resistance_L1L2/RConn1 -- Voltage Measurement/LConn1
  Current Measurement1/RConn1 -- Voltage Measurement1/LConn1 -- Arc_Resistance_L2L3/RConn1
  Current Measurement2/RConn1 -- Voltage Measurement2/LConn1 -- Arc_Resistance_L3L1/RConn1

== system Model_GridElem_Arc_Fault/Arc_Fault/Fault_Model/Cassie_Model/Cassie_Arc_Model/Arc_Equations ==
  enable : Inport
  numberOfArcs : Inport  Port=2
  v_abc : Inport  Port=3
  Enable : EnablePort
  1/T : Gain  Gain=1/Cassie_T
  1/u_0 : Gain  Gain=1/Cassie_V_0
  Add : Sum  Inputs=|+-
  Constant : Constant  Value=(Cassie_G_max-Cassie_G_min)/2
  Constant1 : Constant
  Discrete-Time Integrator : DiscreteIntegrator  ExternalReset=rising  InitialConditionSource=external  SampleTime=-1  LimitOutput=on  UpperSaturationLimit=Cassie_G_max  LowerSaturationLimit=Cassie_G_min  IgnoreLimit=on  ICPrevOutput=DiscIntNeverNeededParam  ICPrevScaledInput=DiscIntNeverNeededParam
  Divide : Product  Inputs=**
  Divide1 : Product  Inputs=**
  Math Function : Math  Operator=square
  Math Function1 : Math  Operator=reciprocal
  R_arc : Outport
  wires:
  Math Function1/1 -> R_arc/1
  v_abc/1 -> 1/u_0/1
  1/u_0/1 -> Math Function/1
  1/T/1 -> Discrete-Time Integrator/1
  enable/1 -> Discrete-Time Integrator/2
  Discrete-Time Integrator/1 -> Divide/2, Math Function1/1
  Math Function/1 -> Add/1
  Constant1/1 -> Add/2
  Add/1 -> Divide/1
  Divide/1 -> 1/T/1
  Divide1/1 -> Discrete-Time Integrator/3
  Constant/1 -> Divide1/1
  numberOfArcs/1 -> Divide1/2

== system Model_GridElem_Arc_Fault/Arc_Fault/Fault_Model/Cassie_Model/Electric_Model/L1G ==
  R_block : Inport
  R_arc : Inport  Port=2
  v_arc : Inport  Port=3
  Add : Sum  Inputs=++|
  Arc_Resistance_L1G : powerlib/Elements/Variable Resistor  Rabsmin=1e-6
  Arc_Voltage_L1G : powerlib/Electrical Sources/Controlled Voltage Source  Initialize=on  Source_Type=AC  Amplitude=0  Phase=0  Frequency=0  Measurements=None
  Constant : Constant
  Current Measurement : powerlib/Measurements/Current Measurement  PhasorSimulation=off  OutputType=Complex  PSBequivalent=0
  Ground{,1..3} (4 alike) : powerlib/Elements/Ground  LConnTagsString=a
  Terminator : Terminator
  Terminator1 : Terminator
  Voltage Measurement : powerlib/Measurements/Voltage Measurement  PhasorSimulation=off  OutputType=Complex  PSBequivalent=0
  Voltage Measurement1 : powerlib/Measurements/Voltage Measurement  PhasorSimulation=off  OutputType=Complex  PSBequivalent=0
  Voltage Measurement2 : powerlib/Measurements/Voltage Measurement  PhasorSimulation=off  OutputType=Complex  PSBequivalent=0
  L1 : PMIOPort  Side=Right
  L2 : PMIOPort  Port=2  Side=Right
  L3 : PMIOPort  Port=3  Side=Right
  numberOfArcs : Outport
  i_arc_meas : Outport  Port=2
  v_arc_meas : Outport  Port=3
  wires:
  Constant/1 -> numberOfArcs/1
  Add/1 -> Arc_Resistance_L1G/1
  R_block/1 -> Add/1
  R_arc/1 -> Add/2
  Voltage Measurement1/1 -> Terminator1/1
  Current Measurement/1 -> i_arc_meas/1
  v_arc/1 -> Arc_Voltage_L1G/1
  Voltage Measurement2/1 -> Terminator/1
  Voltage Measurement/1 -> v_arc_meas/1
  connections:
  Voltage Measurement1/LConn2 -- Ground2/LConn1
  Voltage Measurement1/LConn1 -- L2/RConn1
  Arc_Voltage_L1G/RConn1 -- Arc_Resistance_L1G/LConn1
  Voltage Measurement2/LConn2 -- Ground3/LConn1
  Ground1/LConn1 -- Voltage Measurement/LConn2
  Voltage Measurement2/LConn1 -- L3/RConn1
  Current Measurement/LConn1 -- L1/RConn1
  Ground/LConn1 -- Arc_Voltage_L1G/LConn1
  Voltage Measurement/LConn1 -- Arc_Resistance_L1G/RConn1 -- Current Measurement/RConn1

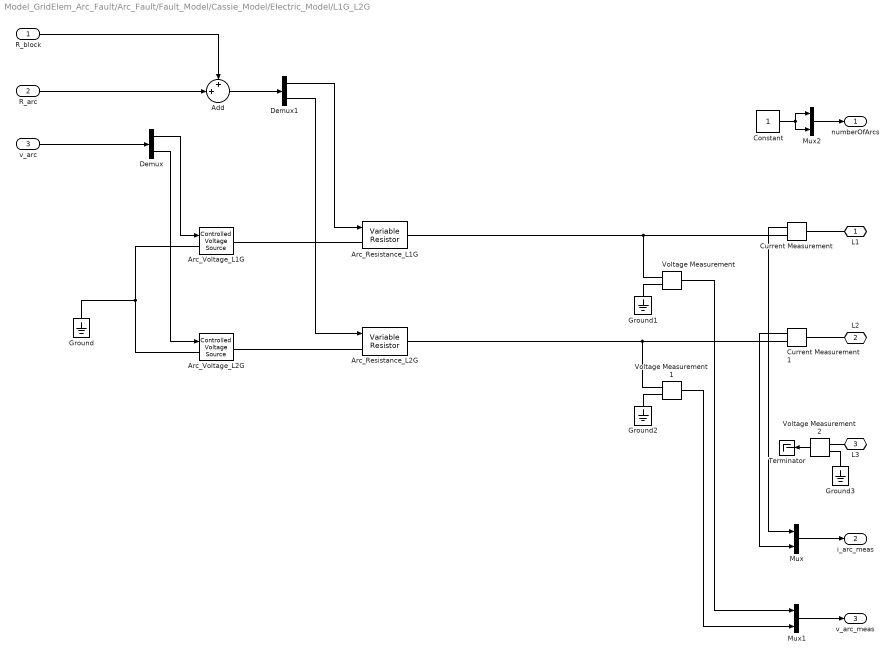
== system Model_GridElem_Arc_Fault/Arc_Fault/Fault_Model/Cassie_Model/Electric_Model/L1G_L2G ==
  R_block : Inport
  R_arc : Inport  Port=2
  v_arc : Inport  Port=3
  Add : Sum  Inputs=++|
  Arc_Resistance_L1G : powerlib/Elements/Variable Resistor  Rabsmin=1e-6
  Arc_Resistance_L2G : powerlib/Elements/Variable Resistor  Rabsmin=1e-6
  Arc_Voltage_L1G : powerlib/Electrical Sources/Controlled Voltage Source  Initialize=on  Source_Type=AC  Amplitude=0  Phase=0  Frequency=0  Measurements=None
  Arc_Voltage_L2G : powerlib/Electrical Sources/Controlled Voltage Source  Initialize=on  Source_Type=AC  Amplitude=0  Phase=0  Frequency=0  Measurements=None
  Constant : Constant
  Current Measurement : powerlib/Measurements/Current Measurement  PhasorSimulation=off  OutputType=Complex  PSBequivalent=0
  Current Measurement1 : powerlib/Measurements/Current Measurement  PhasorSimulation=off  OutputType=Complex  PSBequivalent=0
  Demux : Demux  Outputs=2
  Demux1 : Demux  Outputs=2
  Ground{,1..3} (4 alike) : powerlib/Elements/Ground  LConnTagsString=a
  Mux : Mux  Inputs=2
  Mux1 : Mux  Inputs=2
  Mux2 : Mux  Inputs=2
  Terminator : Terminator
  Voltage Measurement : powerlib/Measurements/Voltage Measurement  PhasorSimulation=off  OutputType=Complex  PSBequivalent=0
  Voltage Measurement1 : powerlib/Measurements/Voltage Measurement  PhasorSimulation=off  OutputType=Complex  PSBequivalent=0
  Voltage Measurement2 : powerlib/Measurements/Voltage Measurement  PhasorSimulation=off  OutputType=Complex  PSBequivalent=0
  L1 : PMIOPort  Side=Right
  L2 : PMIOPort  Port=2  Side=Right
  L3 : PMIOPort  Port=3  Side=Right
  numberOfArcs : Outport
  i_arc_meas : Outport  Port=2
  v_arc_meas : Outport  Port=3
  wires:
  Constant/1 -> Mux2/1, Mux2/2
  Mux2/1 -> numberOfArcs/1
  R_block/1 -> Add/1
  Add/1 -> Demux1/1
  R_arc/1 -> Add/2
  Voltage Measurement2/1 -> Terminator/1
  Voltage Measurement1/1 -> Mux1/2
  Voltage Measurement/1 -> Mux1/1
  Current Measurement1/1 -> Mux/2
  Current Measurement/1 -> Mux/1
  Mux1/1 -> v_arc_meas/1
  Mux/1 -> i_arc_meas/1
  Demux/2 -> Arc_Voltage_L2G/1
  Demux1/2 -> Arc_Resistance_L2G/1
  Demux1/1 -> Arc_Resistance_L1G/1
  v_arc/1 -> Demux/1
  Demux/1 -> Arc_Voltage_L1G/1
  connections:
  Voltage Measurement2/LConn2 -- Ground3/LConn1
  Ground2/LConn1 -- Voltage Measurement1/LConn2
  Ground1/LConn1 -- Voltage Measurement/LConn2
  Current Measurement1/LConn1 -- L2/RConn1
  Voltage Measurement1/LConn1 -- Arc_Resistance_L2G/RConn1 -- Current Measurement1/RConn1
  Current Measurement/LConn1 -- L1/RConn1
  Voltage Measurement/LConn1 -- Arc_Resistance_L1G/RConn1 -- Current Measurement/RConn1
  Arc_Voltage_L1G/RConn1 -- Arc_Resistance_L1G/LConn1
  Arc_Voltage_L2G/RConn1 -- Arc_Resistance_L2G/LConn1
  Voltage Measurement2/LConn1 -- L3/RConn1
  Arc_Voltage_L1G/LConn1 -- Arc_Voltage_L2G/LConn1 -- Ground/LConn1

== system Model_GridElem_Arc_Fault/Arc_Fault/Fault_Model/Cassie_Model/Electric_Model/L1G_L2G_L3G ==
  R_block : Inport
  R_arc : Inport  Port=2
  v_arc : Inport  Port=3
  Add : Sum  Inputs=++|
  Arc_Resistance_L1G : powerlib/Elements/Variable Resistor  Rabsmin=1e-6
  Arc_Resistance_L2G : powerlib/Elements/Variable Resistor  Rabsmin=1e-6
  Arc_Resistance_L3G : powerlib/Elements/Variable Resistor  Rabsmin=1e-6
  Arc_Voltage_L1G : powerlib/Electrical Sources/Controlled Voltage Source  Initialize=on  Source_Type=AC  Amplitude=0  Phase=0  Frequency=0  Measurements=None
  Arc_Voltage_L2G : powerlib/Electrical Sources/Controlled Voltage Source  Initialize=on  Source_Type=AC  Amplitude=0  Phase=0  Frequency=0  Measurements=None
  Arc_Voltage_L3G : powerlib/Electrical Sources/Controlled Voltage Source  Initialize=on  Source_Type=AC  Amplitude=0  Phase=0  Frequency=0  Measurements=None
  Constant : Constant
  Demux : Demux  Outputs=3
  Demux1 : Demux  Outputs=3
  Ground : powerlib/Elements/Ground  LConnTagsString=a
  Mux : Mux  Inputs=3
  Three-Phase V-I Measurement : powerlib/Measurements/Three-Phase V-I Measurement  VoltageMeasurement=phase-to-ground  SetLabelV=off  LabelV=Vabc  Vpu=off  VpuLL=off  CurrentMeasurement=yes  SetLabelI=off  LabelI=Iabc  Ipu=off  Pbase=100e6  Vbase=500e3  OutputType=Complex  PhasorSimulation=off  PSBequivalent=0
  L1 : PMIOPort  Side=Right
  L2 : PMIOPort  Port=2  Side=Right
  L3 : PMIOPort  Port=3  Side=Right
  numberOfArcs : Outport
  i_arc_meas : Outport  Port=2
  v_arc_meas : Outport  Port=3
  wires:
  Constant/1 -> Mux/2, Mux/1, Mux/3
  Mux/1 -> numberOfArcs/1
  R_block/1 -> Add/1
  Add/1 -> Demux1/1
  R_arc/1 -> Add/2
  Demux1/1 -> Arc_Resistance_L1G/1
  Demux1/2 -> Arc_Resistance_L2G/1
  Demux1/3 -> Arc_Resistance_L3G/1
  Demux/1 -> Arc_Voltage_L1G/1
  Demux/2 -> Arc_Voltage_L2G/1
  Demux/3 -> Arc_Voltage_L3G/1
  Three-Phase V-I Measurement/1 -> v_arc_meas/1
  Three-Phase V-I Measurement/2 -> i_arc_meas/1
  v_arc/1 -> Demux/1
  connections:
  Three-Phase V-I Measurement/LConn3 -- L3/RConn1
  Three-Phase V-I Measurement/LConn2 -- L2/RConn1
  Three-Phase V-I Measurement/LConn1 -- L1/RConn1
  Arc_Resistance_L3G/RConn1 -- Three-Phase V-I Measurement/RConn3
  Arc_Resistance_L1G/RConn1 -- Three-Phase V-I Measurement/RConn1
  Ground/LConn1 -- Arc_Voltage_L3G/LConn1 -- Arc_Voltage_L2G/LConn1 -- Arc_Voltage_L1G/LConn1
  Arc_Voltage_L3G/RConn1 -- Arc_Resistance_L3G/LConn1
  Arc_Voltage_L2G/RConn1 -- Arc_Resistance_L2G/LConn1
  Arc_Voltage_L1G/RConn1 -- Arc_Resistance_L1G/LConn1
  Three-Phase V-I Measurement/RConn2 -- Arc_Resistance_L2G/RConn1

== system Model_GridElem_Arc_Fault/Arc_Fault/Fault_Model/Cassie_Model/Electric_Model/L1L2 ==
  R_block : Inport
  R_arc : Inport  Port=2
  v_arc : Inport  Port=3
  Add : Sum  Inputs=++|
  Arc_Resistance_L1L2 : powerlib/Elements/Variable Resistor  Rabsmin=1e-6
  Arc_Voltage_L1L2 : powerlib/Electrical Sources/Controlled Voltage Source  Initialize=on  Source_Type=AC  Amplitude=0  Phase=0  Frequency=0  Measurements=None
  Constant : Constant
  Current Measurement : powerlib/Measurements/Current Measurement  PhasorSimulation=off  OutputType=Complex  PSBequivalent=0
  Ground : powerlib/Elements/Ground  LConnTagsString=a
  Terminator : Terminator
  Voltage Measurement : powerlib/Measurements/Voltage Measurement  PhasorSimulation=off  OutputType=Complex  PSBequivalent=0
  Voltage Measurement1 : powerlib/Measurements/Voltage Measurement  PhasorSimulation=off  OutputType=Complex  PSBequivalent=0
  L1 : PMIOPort  Side=Right
  L2 : PMIOPort  Port=2  Side=Right
  L3 : PMIOPort  Port=3  Side=Right
  numberOfArcs : Outport
  i_arc_meas : Outport  Port=2
  v_arc_meas : Outport  Port=3
  wires:
  Constant/1 -> numberOfArcs/1
  R_block/1 -> Add/1
  Add/1 -> Arc_Resistance_L1L2/1
  R_arc/1 -> Add/2
  Voltage Measurement1/1 -> Terminator/1
  v_arc/1 -> Arc_Voltage_L1L2/1
  Voltage Measurement/1 -> v_arc_meas/1
  Current Measurement/1 -> i_arc_meas/1
  connections:
  Voltage Measurement1/LConn2 -- Ground/LConn1
  Voltage Measurement1/LConn1 -- L3/RConn1
  Arc_Voltage_L1L2/RConn1 -- Arc_Resistance_L1L2/LConn1
  Current Measurement/LConn1 -- L1/RConn1
  L2/RConn1 -- Arc_Voltage_L1L2/LConn1 -- Voltage Measurement/LConn2
  Voltage Measurement/LConn1 -- Arc_Resistance_L1L2/RConn1 -- Current Measurement/RConn1

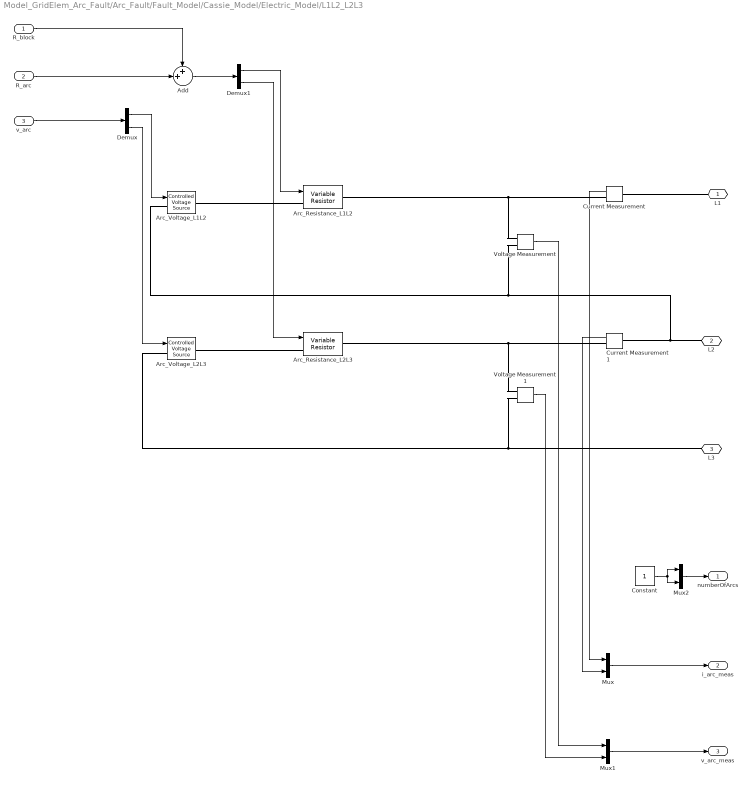
== system Model_GridElem_Arc_Fault/Arc_Fault/Fault_Model/Cassie_Model/Electric_Model/L1L2_L2L3 ==
  R_block : Inport
  R_arc : Inport  Port=2
  v_arc : Inport  Port=3
  Add : Sum  Inputs=++|
  Arc_Resistance_L1L2 : powerlib/Elements/Variable Resistor  Rabsmin=1e-6
  Arc_Resistance_L2L3 : powerlib/Elements/Variable Resistor  Rabsmin=1e-6
  Arc_Voltage_L1L2 : powerlib/Electrical Sources/Controlled Voltage Source  Initialize=on  Source_Type=AC  Amplitude=0  Phase=0  Frequency=0  Measurements=None
  Arc_Voltage_L2L3 : powerlib/Electrical Sources/Controlled Voltage Source  Initialize=on  Source_Type=AC  Amplitude=0  Phase=0  Frequency=0  Measurements=None
  Constant : Constant
  Current Measurement : powerlib/Measurements/Current Measurement  PhasorSimulation=off  OutputType=Complex  PSBequivalent=0
  Current Measurement1 : powerlib/Measurements/Current Measurement  PhasorSimulation=off  OutputType=Complex  PSBequivalent=0
  Demux : Demux  Outputs=2
  Demux1 : Demux  Outputs=2
  Mux : Mux  Inputs=2
  Mux1 : Mux  Inputs=2
  Mux2 : Mux  Inputs=2
  Voltage Measurement : powerlib/Measurements/Voltage Measurement  PhasorSimulation=off  OutputType=Complex  PSBequivalent=0
  Voltage Measurement1 : powerlib/Measurements/Voltage Measurement  PhasorSimulation=off  OutputType=Complex  PSBequivalent=0
  L1 : PMIOPort  Side=Right
  L2 : PMIOPort  Port=2  Side=Right
  L3 : PMIOPort  Port=3  Side=Right
  numberOfArcs : Outport
  i_arc_meas : Outport  Port=2
  v_arc_meas : Outport  Port=3
  wires:
  Constant/1 -> Mux2/1, Mux2/2
  Mux2/1 -> numberOfArcs/1
  R_block/1 -> Add/1
  R_arc/1 -> Add/2
  Add/1 -> Demux1/1
  Demux1/2 -> Arc_Resistance_L2L3/1
  Voltage Measurement1/1 -> Mux1/2
  Voltage Measurement/1 -> Mux1/1
  Demux/2 -> Arc_Voltage_L2L3/1
  Demux1/1 -> Arc_Resistance_L1L2/1
  Mux1/1 -> v_arc_meas/1
  Demux/1 -> Arc_Voltage_L1L2/1
  v_arc/1 -> Demux/1
  Current Measurement1/1 -> Mux/2
  Mux/1 -> i_arc_meas/1
  Current Measurement/1 -> Mux/1
  connections:
  Arc_Voltage_L1L2/RConn1 -- Arc_Resistance_L1L2/LConn1
  Arc_Voltage_L2L3/RConn1 -- Arc_Resistance_L2L3/LConn1
  Voltage Measurement1/LConn1 -- Arc_Resistance_L2L3/RConn1 -- Current Measurement1/RConn1
  Arc_Voltage_L1L2/LConn1 -- L2/RConn1 -- Current Measurement1/LConn1 -- Voltage Measurement/LConn2
  L3/RConn1 -- Arc_Voltage_L2L3/LConn1 -- Voltage Measurement1/LConn2
  Voltage Measurement/LConn1 -- Arc_Resistance_L1L2/RConn1 -- Current Measurement/RConn1
  Current Measurement/LConn1 -- L1/RConn1
